simulink model "HoverLock"  (R2024b)
settings: Solver=ode15s  StartTime=0.0  StopTime=8  FixedStep=1/120  MaxStep=0.01  RelTol=1e-1
PreLoadFcn:
  | [aircraft, state] = astDehavillandBeaver();
  | thrustX = getCoefficient(aircraft,"CX","Propeller",Component="Propeller");
model workspace (MATLAB code in the model file + MAT data in the model file):
  inputs0.time = 0
  inputs0.signals(1).dimensions = 1
  inputs0.signals(1).values = -0.104711430294
  inputs0.signals(2).dimensions = 1
  inputs0.signals(2).values = -0.0698725229544
  inputs0.signals(3).dimensions = 1
  inputs0.signals(3).values = -0.000215042330254
  states.time = 0
  states.signals(1).values = 0
  states.signals(1).dimensions = 1
  states.signals(1).label = 'CSTATE'
  states.signals(1).blockName = 'asb6DOFAirframeTemplate/6DOF EOM/6DOF (Euler Angles)/xe,ye,ze'
  states.signals(1).stateName = 'Xe'
  states.signals(1).inReferencedModel = 0
  states.signals(1).sampleTime = [0 0]
  states.signals(2).values = 0
  states.signals(2).dimensions = 1
  states.signals(2).label = 'CSTATE'
  states.signals(2).blockName = 'asb6DOFAirframeTemplate/6DOF EOM/6DOF (Euler Angles)/xe,ye,ze'
  states.signals(2).stateName = 'Ye'
  states.signals(2).inReferencedModel = 0
  states.signals(2).sampleTime = [0 0]
  states.signals(3).values = -2202
  states.signals(3).dimensions = 1
  states.signals(3).label = 'CSTATE'
  states.signals(3).blockName = 'asb6DOFAirframeTemplate/6DOF EOM/6DOF (Euler Angles)/xe,ye,ze'
  states.signals(3).stateName = 'Ze'
  states.signals(3).inReferencedModel = 0
  states.signals(3).sampleTime = [0 0]
  states.signals(4).values = 0.128665353089
  states.signals(4).dimensions = 1
  states.signals(4).label = 'CSTATE'
  states.signals(4).blockName = 'asb6DOFAirframeTemplate/6DOF EOM/6DOF (Euler Angles)/Calculate DCM &
    | Euler Angles/phi
    | theta
    | psi'
  states.signals(4).stateName = 'phi'
  states.signals(4).inReferencedModel = 0
  states.signals(4).sampleTime = [0 0]
  states.signals(5).values = 0.259337659946
  states.signals(5).dimensions = 1
  states.signals(5).label = 'CSTATE'
  states.signals(5).blockName = 'asb6DOFAirframeTemplate/6DOF EOM/6DOF (Euler Angles)/Calculate DCM &
    | Euler Angles/phi
    | theta
    | psi'
  states.signals(5).stateName = 'theta'
  states.signals(5).inReferencedModel = 0
  states.signals(5).sampleTime = [0 0]
  states.signals(6).values = -0.178947917154
  states.signals(6).dimensions = 1
  states.signals(6).label = 'CSTATE'
  states.signals(6).blockName = 'asb6DOFAirframeTemplate/6DOF EOM/6DOF (Euler Angles)/Calculate DCM &
    | Euler Angles/phi
    | theta
    | psi'
  states.signals(6).stateName = 'psi'
  states.signals(6).inReferencedModel = 0
  states.signals(6).sampleTime = [0 0]
  states.signals(7).values = 36.9119692666
  states.signals(7).dimensions = 1
  states.signals(7).label = 'CSTATE'
  states.signals(7).blockName = 'asb6DOFAirframeTemplate/6DOF EOM/6DOF (Euler Angles)/ub,vb,wb'
  states.signals(7).stateName = 'Ubody'
  states.signals(7).inReferencedModel = 0
  states.signals(7).sampleTime = [0 0]
  states.signals(8).values = 8.10720863264
  states.signals(8).dimensions = 1
  states.signals(8).label = 'CSTATE'
  states.signals(8).blockName = 'asb6DOFAirframeTemplate/6DOF EOM/6DOF (Euler Angles)/ub,vb,wb'
  states.signals(8).stateName = 'Vbody'
  states.signals(8).inReferencedModel = 0
  states.signals(8).sampleTime = [0 0]
  states.signals(9).values = 8.82591882596
  states.signals(9).dimensions = 1
  states.signals(9).label = 'CSTATE'
  states.signals(9).blockName = 'asb6DOFAirframeTemplate/6DOF EOM/6DOF (Euler Angles)/ub,vb,wb'
  states.signals(9).stateName = 'Wbody'
  states.signals(9).inReferencedModel = 0
  states.signals(9).sampleTime = [0 0]
  states.signals(10).values = 0
  states.signals(10).dimensions = 1
  states.signals(10).label = 'CSTATE'
  states.signals(10).blockName = 'asb6DOFAirframeTemplate/6DOF EOM/6DOF (Euler Angles)/p,q,r '
  states.signals(10).stateName = 'p'
  states.signals(10).inReferencedModel = 0
  states.signals(10).sampleTime = [0 0]
  states.signals(11).values = 0
  states.signals(11).dimensions = 1
  states.signals(11).label = 'CSTATE'
  states.signals(11).blockName = 'asb6DOFAirframeTemplate/6DOF EOM/6DOF (Euler Angles)/p,q,r '
  states.signals(11).stateName = 'q'
  states.signals(11).inReferencedModel = 0
  states.signals(11).sampleTime = [0 0]
  states.signals(12).values = 0
  states.signals(12).dimensions = 1
  states.signals(12).label = 'CSTATE'
  states.signals(12).blockName = 'asb6DOFAirframeTemplate/6DOF EOM/6DOF (Euler Angles)/p,q,r '
  states.signals(12).stateName = 'r'
  states.signals(12).inReferencedModel = 0
  states.signals(12).sampleTime = [0 0]
  states.signals(13).values = [0 0]
  states.signals(13).dimensions = 2
  states.signals(13).label = 'CSTATE'
  states.signals(13).blockName = 'asb6DOFAirframeTemplate/Environment Model/Dryden Wind Turbulence Model 
    | (Continuous (+q +r))/Filters on velocities/Hwgw(s)/wg_p1'
  states.signals(13).stateName = ''
  states.signals(13).inReferencedModel = 0
  states.signals(13).sampleTime = [0 0]
  states.signals(14).values = [0 0]
  states.signals(14).dimensions = 2
  states.signals(14).label = 'CSTATE'
  states.signals(14).blockName = 'asb6DOFAirframeTemplate/Environment Model/Dryden Wind Turbulence Model 
    | (Continuous (+q +r))/Filters on velocities/Hwgw(s)/wg_p2'
  states.signals(14).stateName = ''
  states.signals(14).inReferencedModel = 0
  states.signals(14).sampleTime = [0 0]
  states.signals(15).values = [0 0]
  states.signals(15).dimensions = 2
  states.signals(15).label = 'CSTATE'
  states.signals(15).blockName = 'asb6DOFAirframeTemplate/Environment Model/Dryden Wind Turbulence Model 
    | (Continuous (+q +r))/Filters on velocities/Hvgw(s)/vg_p1'
  states.signals(15).stateName = ''
  states.signals(15).inReferencedModel = 0
  states.signals(15).sampleTime = [0 0]
  states.signals(16).values = [0 0]
  states.signals(16).dimensions = 2
  states.signals(16).label = 'CSTATE'
  states.signals(16).blockName = 'asb6DOFAirframeTemplate/Environment Model/Dryden Wind Turbulence Model 
    | (Continuous (+q +r))/Filters on velocities/Hvgw(s)/vgw_p2'
  states.signals(16).stateName = ''
  states.signals(16).inReferencedModel = 0
  states.signals(16).sampleTime = [0 0]
  states.signals(17).values = [0 0]
  states.signals(17).dimensions = 2
  states.signals(17).label = 'CSTATE'
  states.signals(17).blockName = 'asb6DOFAirframeTemplate/Environment Model/Dryden Wind Turbulence Model 
    | (Continuous (+q +r))/Filters on velocities/Hugw(s)/ug_p'
  states.signals(17).stateName = ''
  states.signals(17).inReferencedModel = 0
  states.signals(17).sampleTime = [0 0]
  states.signals(18).values = [0 0]
  states.signals(18).dimensions = 2
  states.signals(18).label = 'CSTATE'
  states.signals(18).blockName = 'asb6DOFAirframeTemplate/Environment Model/Dryden Wind Turbulence Model 
    | (Continuous (+q +r))/Filters on angular rates/Hrgw/rgw_p'
  states.signals(18).stateName = ''
  states.signals(18).inReferencedModel = 0
  states.signals(18).sampleTime = [0 0]
  states.signals(19).values = [0 0]
  states.signals(19).dimensions = 2
  states.signals(19).label = 'CSTATE'
  states.signals(19).blockName = 'asb6DOFAirframeTemplate/Environment Model/Dryden Wind Turbulence Model 
    | (Continuous (+q +r))/Filters on angular rates/Hqgw/qgw_p'
  states.signals(19).stateName = ''
  states.signals(19).inReferencedModel = 0
  states.signals(19).sampleTime = [0 0]
  states.signals(20).values = [0 0]
  states.signals(20).dimensions = 2
  states.signals(20).label = 'CSTATE'
  states.signals(20).blockName = 'asb6DOFAirframeTemplate/Environment Model/Dryden Wind Turbulence Model 
    | (Continuous (+q +r))/Filters on angular rates/Hpgw/pgw_p'
  states.signals(20).stateName = ''
  states.signals(20).inReferencedModel = 0
  states.signals(20).sampleTime = [0 0]
  states0.time = 0
  states0.signals(1).values = [0 0 -2202]
  states0.signals(1).dimensions = 3
  states0.signals(1).label = 'CSTATE'
  states0.signals(1).blockName = 'asb6DOFAirframeTemplate/6DOF EOM/6DOF (Euler Angles)/xe,ye,ze'
  states0.signals(1).stateName = ''
  states0.signals(1).inReferencedModel = 0
  states0.signals(1).sampleTime = [0 0]
  states0.signals(2).values = [0.128665353089 0.259337659946 -0.178947917154]
  states0.signals(2).dimensions = 3
  states0.signals(2).label = 'CSTATE'
  states0.signals(2).blockName = 'asb6DOFAirframeTemplate/6DOF EOM/6DOF (Euler Angles)/Calculate DCM &
    | Euler Angles/phi
    | theta
    | psi'
  states0.signals(2).stateName = ''
  states0.signals(2).inReferencedModel = 0
  states0.signals(2).sampleTime = [0 0]
  states0.signals(3).values = [36.9119692666 8.10720863264 8.82591882596]
  states0.signals(3).dimensions = 3
  states0.signals(3).label = 'CSTATE'
  states0.signals(3).blockName = 'asb6DOFAirframeTemplate/6DOF EOM/6DOF (Euler Angles)/ub,vb,wb'
  states0.signals(3).stateName = ''
  states0.signals(3).inReferencedModel = 0
  states0.signals(3).sampleTime = [0 0]
  states0.signals(4).values = [0 0 0]
  states0.signals(4).dimensions = 3
  states0.signals(4).label = 'CSTATE'
  states0.signals(4).blockName = 'asb6DOFAirframeTemplate/6DOF EOM/6DOF (Euler Angles)/p,q,r '
  states0.signals(4).stateName = ''
  states0.signals(4).inReferencedModel = 0
  states0.signals(4).sampleTime = [0 0]
  states0.signals(5).values = [0 0]
  states0.signals(5).dimensions = 2
  states0.signals(5).label = 'CSTATE'
  states0.signals(5).blockName = 'asb6DOFAirframeTemplate/Environment Model/Dryden Wind Turbulence Model 
    | (Continuous (+q +r))/Filters on velocities/Hwgw(s)/wg_p1'
  states0.signals(5).stateName = ''
  states0.signals(5).inReferencedModel = 0
  states0.signals(5).sampleTime = [0 0]
  states0.signals(6).values = [0 0]
  states0.signals(6).dimensions = 2
  states0.signals(6).label = 'CSTATE'
  states0.signals(6).blockName = 'asb6DOFAirframeTemplate/Environment Model/Dryden Wind Turbulence Model 
    | (Continuous (+q +r))/Filters on velocities/Hwgw(s)/wg_p2'
  states0.signals(6).stateName = ''
  states0.signals(6).inReferencedModel = 0
  states0.signals(6).sampleTime = [0 0]
  states0.signals(7).values = [0 0]
  states0.signals(7).dimensions = 2
  states0.signals(7).label = 'CSTATE'
  states0.signals(7).blockName = 'asb6DOFAirframeTemplate/Environment Model/Dryden Wind Turbulence Model 
    | (Continuous (+q +r))/Filters on velocities/Hvgw(s)/vg_p1'
  states0.signals(7).stateName = ''
  states0.signals(7).inReferencedModel = 0
  states0.signals(7).sampleTime = [0 0]
  states0.signals(8).values = [0 0]
  states0.signals(8).dimensions = 2
  states0.signals(8).label = 'CSTATE'
  states0.signals(8).blockName = 'asb6DOFAirframeTemplate/Environment Model/Dryden Wind Turbulence Model 
    | (Continuous (+q +r))/Filters on velocities/Hvgw(s)/vgw_p2'
  states0.signals(8).stateName = ''
  states0.signals(8).inReferencedModel = 0
  states0.signals(8).sampleTime = [0 0]
  states0.signals(9).values = [0 0]
  states0.signals(9).dimensions = 2
  states0.signals(9).label = 'CSTATE'
  states0.signals(9).blockName = 'asb6DOFAirframeTemplate/Environment Model/Dryden Wind Turbulence Model 
    | (Continuous (+q +r))/Filters on velocities/Hugw(s)/ug_p'
  states0.signals(9).stateName = ''
  states0.signals(9).inReferencedModel = 0
  states0.signals(9).sampleTime = [0 0]
  states0.signals(10).values = [0 0]
  states0.signals(10).dimensions = 2
  states0.signals(10).label = 'CSTATE'
  states0.signals(10).blockName = 'asb6DOFAirframeTemplate/Environment Model/Dryden Wind Turbulence Model 
    | (Continuous (+q +r))/Filters on angular rates/Hrgw/rgw_p'
  states0.signals(10).stateName = ''
  states0.signals(10).inReferencedModel = 0
  states0.signals(10).sampleTime = [0 0]
  states0.signals(11).values = [0 0]
  states0.signals(11).dimensions = 2
  states0.signals(11).label = 'CSTATE'
  states0.signals(11).blockName = 'asb6DOFAirframeTemplate/Environment Model/Dryden Wind Turbulence Model 
    | (Continuous (+q +r))/Filters on angular rates/Hqgw/qgw_p'
  states0.signals(11).stateName = ''
  states0.signals(11).inReferencedModel = 0
  states0.signals(11).sampleTime = [0 0]
  states0.signals(12).values = [0 0]
  states0.signals(12).dimensions = 2
  states0.signals(12).label = 'CSTATE'
  states0.signals(12).blockName = 'asb6DOFAirframeTemplate/Environment Model/Dryden Wind Turbulence Model 
    | (Continuous (+q +r))/Filters on angular rates/Hpgw/pgw_p'
  states0.signals(12).stateName = ''
  states0.signals(12).inReferencedModel = 0
  states0.signals(12).sampleTime = [0 0]
  other statements: initialize6DOFSkyHogg;
libraries: fl_lib x15, slpidlib x10, nesl_utility x3, simulink x3
settings Model: Creator=asus  LastModifiedBy=asus
settings SolverCC: AlgebraicLoopSolver=TrustRegion  AutoInsertRateTranBlk=on  InsertRTBMode=Never (minimum delay)  MinimalZcImpactIntegration=on  MaxZcPerStep=1
settings DataIOCC: ExternalInput=inputs0  InitialState=states  SaveFormat=Array  SaveOutput=off
settings OptimizationCC: EnhancedBackFolding=on  StrengthReduction=on  InitFltsAndDblsToZero=on  DifferentSizesBufferReuse=on
settings DebuggingCC: WriteAfterWriteMsg=DisableAll  AlgebraicLoopMsg=none  FcnCallInpInsideContextMsg=warning  UniqueDataStoreMsg=error  RootOutportRequireBusObject=none  StateNameClashWarn=warning  StrictBusMsg=ErrorOnBusTreatedAsVector  SFUnexpectedBacktrackingDiag=warning  SFNoUnconditionalDefaultTransitionDiag=warning  SFExecutionAtInitializationDiag=none  ArithmeticOperatorsInVariantConditions=warning
settings ModelReferenceCC: EnableRefExpFcnMdlSchedulingChecks=on  PropagateSignalLabelsOutOfModel=off
settings SFSimCC: SimUseLocalCustomCode=off
settings RTWCC: RTWUseLocalCustomCode=off  GPUComputeCapability=3.5  DLArmComputeVersion=19.05
settings CodeAppCC: StateflowObjectComments=on

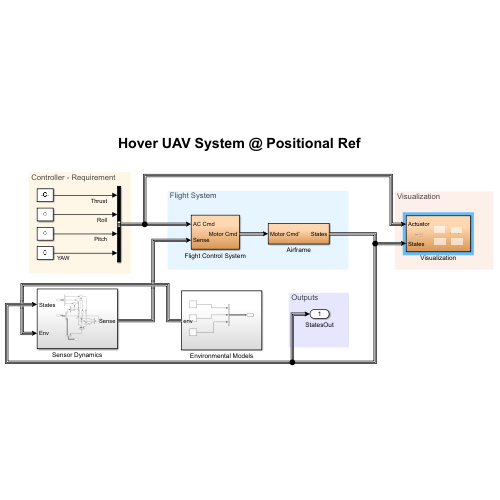
[thumbnail: Simulink's stored preview of the top-level diagram]
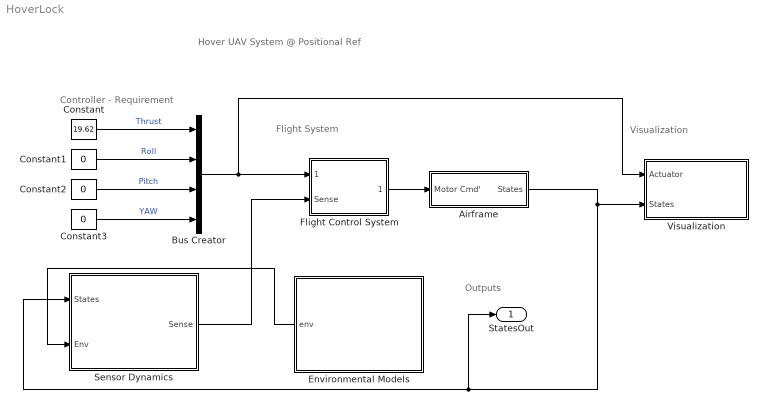
== system HoverLock ==
  note: Hover UAV System @ Positional Ref
  note: Flight System
  note: Controller - Requirement
  note: Visualization
  note: Outputs
  Airframe : Subsystem  VariantControl=eom3DOF
  Bus Creator : BusCreator  Inputs=4
  Constant : Constant  Value=19.62
  Constant1 : Constant  Value=0
  Constant2 : Constant  Value=0
  Constant3 : Constant  Value=0
  Environmental Models : Subsystem
  Flight Control System : Subsystem  VariantControl=aeroCONST
  Sensor Dynamics : Subsystem
  Visualization : Subsystem
  StatesOut : Outport  OutDataTypeStr=double  VectorParamsAs1DForOutWhenUnconnected=off
  wires:
  Constant/1 -> Bus Creator/1  "Thrust"
  Constant1/1 -> Bus Creator/2  "Roll"
  Constant2/1 -> Bus Creator/3  "Pitch"
  Airframe/1(States) -> Visualization/2(States), StatesOut/1, Sensor Dynamics/1(States)
  Environmental Models/1(env) -> Sensor Dynamics/2(Env)
  Constant3/1 -> Bus Creator/4  "YAW"
  Bus Creator/1 -> Visualization/1(Actuator), Flight Control System/1(AC Cmd)
  Flight Control System/1(Motor Cmd) -> Airframe/1(Motor Cmd')
  Sensor Dynamics/1(Sense) -> Flight Control System/2(Sense)

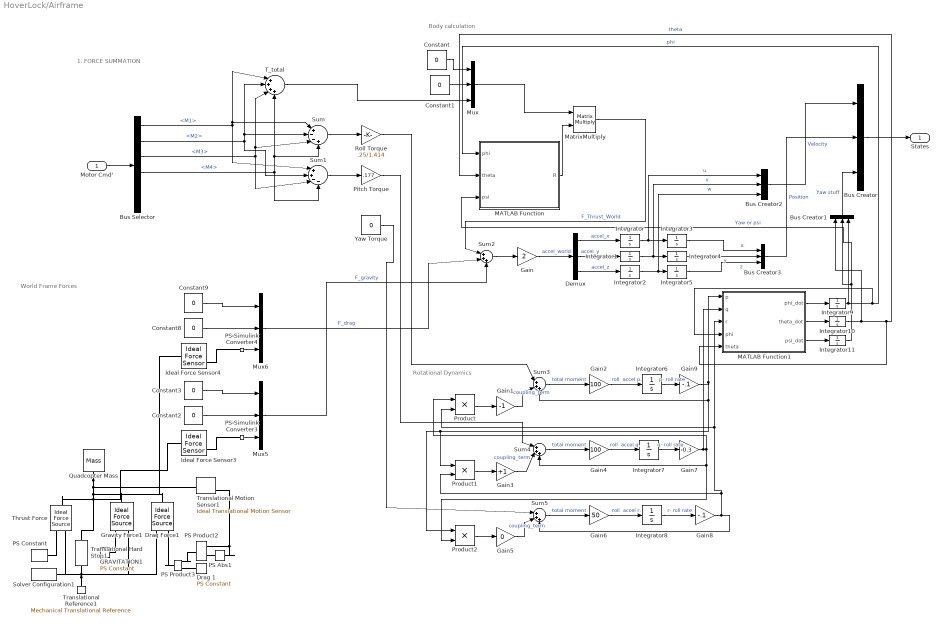
== system HoverLock/Airframe ==
  note: Body calculation
  note: Rotational Dynamics
  note: World Frame Forces
  note: 1. FORCE SUMMATION
  Motor Cmd' : Inport
  Bus Creator{,1..3} (4 alike) : BusCreator  Inputs=3
  Bus Selector : BusSelector  OutputSignals=M1,M2,M3,M4,theta,phi
  Constant : Constant  Value=0  VectorParams1D=off
  Constant1 : Constant  Value=0  VectorParams1D=off
  Constant{2..3,8..9} (4 alike) : Constant  Value=0
  Demux : Demux  Outputs=3
  Drag Force1 : fl_lib/Mechanical/Mechanical Sources/Ideal Force Source
  Drag 1 : fl_lib/Physical Signals/Sources/PS Constant  constant=-.5*1.225*1.1*0.006 N/(m/s)^2
  GRAVITATION1 : fl_lib/Physical Signals/Sources/PS Constant  constant=-9.81*.07 N
  Gain : Gain  Gain=2
  Gain1 : Gain  Gain=-1
  Gain2 : Gain  Gain=100
  Gain3 : Gain  Gain=+1
  Gain4 : Gain  Gain=100
  Gain5 : Gain  Gain=0
  Gain6 : Gain  Gain=50
  Gain7 : Gain  Gain=-0.3
  Gain8 : Gain  Gain=-.1
  Gain9 : Gain  Gain=-.1
  Gravity Force1 : fl_lib/Mechanical/Mechanical Sources/Ideal Force Source
  Ideal Force Sensor3 : fl_lib/Mechanical/Mechanical Sensors/Ideal Force Sensor
  Ideal Force Sensor4 : fl_lib/Mechanical/Mechanical Sensors/Ideal Force Sensor
  Integrator{,1..4,6..11} (11 alike) : Integrator
  Integrator5 : Integrator  InitialCondition=1
  MATLAB Function : MATLAB Function  TreatAsAtomicUnit=on
  MATLAB Function1 : MATLAB Function  TreatAsAtomicUnit=on
  MatrixMultiply : Product  Multiplication=Matrix(*)
  Mux : Mux  Inputs=3
  Mux5 : Mux  Inputs=3
  Mux6 : Mux  Inputs=3
  PS Abs1 : fl_lib/Physical Signals/Nonlinear Operators/PS Abs
      settings: InternalSimscapePortConfiguration="{\"Bottom\":[],\"Left\":[{\"id\":\"I\",\"label\":\"\",\"type\":\"input\"}],\"Right\":[{\"id\":\"O\",\"label\":\"\",\"type\":\"output\"}],\"Top\":[]}"
  PS Constant : fl_lib/Physical Signals/Sources/PS Constant  constant=19.62 N
  PS Product2 : fl_lib/Physical Signals/Functions/PS Product
  PS Product3 : fl_lib/Physical Signals/Functions/PS Product
  PS-Simulink Converter3 : nesl_utility/PS-Simulink Converter  PhysicalDomain=network_engine_domain  SubClassName=ps_output  LeftPortType=input  RightPortType=output  PseudoPeriodic=off  Frequencies=[]  VectorFormat=inherit  Unit=inherit  AffineConversion=off
  PS-Simulink Converter4 : nesl_utility/PS-Simulink Converter  PhysicalDomain=network_engine_domain  SubClassName=ps_output  LeftPortType=input  RightPortType=output  PseudoPeriodic=off  Frequencies=[]  VectorFormat=inherit  Unit=inherit  AffineConversion=off
  Pitch Torque : Gain  Gain=.177
  Product : Product
  Product1 : Product
  Product2 : Product
  Quadcopter Mass : fl_lib/Mechanical/Translational Elements/Mass  mass=.07 kg  num_ports=foundation.enum.numPorts2.one  v_specify=off  v_priority=High  v=0 m/s  v_nominal_specify=off  v_nominal_value=1  v_nominal_unit=m/s  f_specify=off  f_priority=None  f=0 N  f_nominal_specify=off  f_nominal_value=1  f_nominal_unit=N
  Roll Torque : Gain  Gain=.25/1.414
  Solver Configuration1 : nesl_utility/Solver Configuration  PhysicalDomain=network_engine_domain  SubClassName=solver  LeftPortType=input  RightPortType=generic  Tones=[]  Harmonics=[]  SimulateNoise=off  Profile=off  UseLocalSampling=off  EnableSwitchedLinearOptims=on  FrequencyDomain=off  UseCCode=off  RelTol=0.001  AbsTol=0.001  MinStep=1e-09  ToWorkspace=off  RevertToSquareIcSolve=off  NumHomotopyIterations=100  PhasorMode=off  PhasorModeNumHarmonics=1  ConsistencySolver=NEWTON_XTOL_AFTER_FTOL  IndexReductionMethod=DerivativeReplacement  DoDC=off  ResidualTolerance=1e-09  ConsistencyTolSource=GLOBAL  ConsistencyAbsTol=0.001  ConsistencyRelTol=0.001  ConsistencyTolFactor=0.001  UseLocalSolver=off  LocalSolverChoice=NE_BACKWARD_EULER_ADVANCER  ResolveIndetEquations=on  FunctionEvalNumThread=1  LocalSolverSampleTime=0.001  DoFixedCost=off  MaxNonlinIter=3  MaxModeIter=2  ComputeImpulses=off  ImpulseIterations=2  LinearAlgebra=auto  LinearAlgebraNumThread=0  EquationFormulation=NE_TIME_EF  DelaysMemoryBudget=1024  AutomaticFiltering=on  FilteringTimeConstant=0.001  PartitionStorageMethod=AS_NEEDED  PartitionMemoryBudget=1024  PartitionMethod=ROBUST  MultibodyUseLocalSolver=off  MultibodyLocalSolverChoice=ODE1  MultibodyLocalSolverSampleTime=0.001
  Sum : Sum  Inputs=|+--+
  Sum1 : Sum  Inputs=|++--
  Sum{2..5} (4 alike) : Sum  Inputs=|+++
  T_total : Sum  Inputs=|++++
  Thrust Force : fl_lib/Mechanical/Mechanical Sources/Ideal Force Source
  Translational Motion Sensor1 : fl_lib/Mechanical/Mechanical Sensors/Ideal Translational Motion Sensor  reference=foundation.enum.MeasurementReference.absolute  acceleration_port=false  velocity_port=true  position_port=true  offset=0 m
      settings: InternalSimscapePortConfiguration="{\"Bottom\":[],\"Left\":[{\"id\":\"R\",\"label\":\"R\",\"type\":\"foundation.mechanical.translational.translational\"}],\"Right\":[{\"id\":\"V\",\"label\":\"V\",\"type\":\"output\"},{\"id\":\"P\",\"label\":\"P\",\"type\":\"output\"}],\"Top\":[]}"
  Translational Reference1 : fl_lib/Mechanical/Translational Elements/Mechanical Translational Reference
  Translational Hard Stop1 : fl_lib/Mechanical/Translational Elements/Translational Hard Stop  upper_bnd=inf m  lower_bnd=0 m  model=simscape.enum.hardstop.smooth  stiff_up=1e6 N/m  stiff_low=270 N/m  D_up=150 N*s/m  D_low=150 N*s/m  transition=0.1 mm  coeff_rest=0.7  v_tol=0.001 m/s  f_tol=0.001 N  v_specify=off  v_priority=None  v=0 m/s  v_nominal_specify=off  v_nominal_value=1  v_nominal_unit=m/s  f_specify=off  f_priority=None  f=0 N  f_nominal_specify=off  f_nominal_value=1  f_nominal_unit=N  x_specify=off  x_priority=High  x=0 m  x_nominal_specify=off  x_nominal_value=1  x_nominal_unit=m  M_specify=off  M_priority=None  M=0
  Yaw Torque : Constant  Value=0
  States : Outport
  wires:
  Motor Cmd'/1 -> Bus Selector/1
  Bus Selector/2 -> Sum/2, T_total/2, Sum1/2  "<M2>"
  Bus Selector/3 -> Sum1/3, T_total/3, Sum/3  "<M3>"
  Bus Selector/4 -> Sum1/4, Sum/4, T_total/4  "<M4>"
  Bus Selector/1 -> Sum/1, T_total/1, Sum1/1  "<M1>"
  Sum/1 -> Roll Torque/1
  Sum1/1 -> Pitch Torque/1
  Constant/1 -> Mux/1
  Constant1/1 -> Mux/2
  T_total/1 -> Mux/3
  Mux/1 -> MatrixMultiply/1
  MATLAB Function/1(R) -> MatrixMultiply/2
  MatrixMultiply/1 -> Sum2/1  "F_Thrust_World"
  Sum2/1 -> Gain/1
  Gain/1 -> Demux/1  "accel_world"
  Demux/1 -> Integrator/1  "accel_x"
  Demux/2 -> Integrator1/1  "accel_y"
  Demux/3 -> Integrator2/1  "accel_z"
  Integrator/1 -> Bus Creator2/1, Integrator3/1  "u"
  Integrator1/1 -> Bus Creator2/2, Integrator4/1  "v"
  Integrator2/1 -> Bus Creator2/3, Integrator5/1  "w"
  Integrator3/1 -> Bus Creator3/1  "x"
  Integrator4/1 -> Bus Creator3/2  "y"
  Integrator5/1 -> Bus Creator3/3  "z"
  Product/1 -> Gain1/1
  Gain1/1 -> Sum3/2  "coupling_term"
  Sum3/1 -> Gain2/1  "total moment"
  Gain2/1 -> Integrator6/1  "roll  accel p."
  Integrator6/1 -> Gain9/1  "p- roll rate"
  Sum4/1 -> Gain4/1  "total moment"
  Gain3/1 -> Sum4/2  "coupling_term"
  Product1/1 -> Gain3/1
  Product2/1 -> Gain5/1
  Gain5/1 -> Sum5/2  "coupling_term"
  Sum5/1 -> Gain6/1  "total moment"
  Gain6/1 -> Integrator8/1  "roll  accel r."
  Integrator8/1 -> Gain8/1  "r- roll rate"
  Roll Torque/1 -> Sum3/1
  Pitch Torque/1 -> Sum4/1
  Yaw Torque/1 -> Sum5/1
  MATLAB Function1/1(phi_dot) -> Integrator9/1
  MATLAB Function1/2(theta_dot) -> Integrator10/1
  MATLAB Function1/3(psi_dot) -> Integrator11/1
  Integrator9/1 -> MATLAB Function1/4(phi), MATLAB Function/1(phi), Bus Creator1/3  "phi"
  Integrator10/1 -> Bus Creator1/1, MATLAB Function1/5(theta), MATLAB Function/2(theta)  "theta"
  Integrator11/1 -> Bus Creator1/2, MATLAB Function/3(psi)  "Yaw or psi"
  Bus Creator/1 -> States/1
  Bus Creator1/1 -> Bus Creator/3  "Yaw stuff"
  Gain7/1 -> Product2/2, Sum4/3, Product/1, MATLAB Function1/2(q)
  Integrator7/1 -> Gain7/1  "q- roll rate"
  Gain8/1 -> Sum5/3, Product1/2, Product/2, MATLAB Function1/3(r)
  Gain9/1 -> Product2/1, Product1/1, Sum3/3, MATLAB Function1/1(p)
  Gain4/1 -> Integrator7/1  "roll  accel q."
  Constant8/1 -> Mux6/2
  Mux6/1 -> Sum2/2  "F_drag"
  PS-Simulink Converter4/1 -> Mux6/3
  Constant9/1 -> Mux6/1
  Constant3/1 -> Mux5/1
  PS-Simulink Converter3/1 -> Mux5/3
  Constant2/1 -> Mux5/2
  Mux5/1 -> Sum2/3  "F_gravity"
  Bus Creator2/1 -> Bus Creator/1  "Velocity"
  Bus Creator3/1 -> Bus Creator/2  "Position"
  connections:
  Translational Reference1/LConn1 -- Drag Force1/RConn2 -- Gravity Force1/RConn2 -- Translational Hard Stop1/RConn1 -- Thrust Force/RConn2 -- Solver Configuration1/RConn1
  PS Abs1/LConn1 -- Translational Motion Sensor1/RConn1 -- PS Product2/LConn1
  Quadcopter Mass/LConn1 -- Translational Motion Sensor1/LConn1 -- Ideal Force Sensor4/LConn1 -- Drag Force1/LConn1 -- Ideal Force Sensor3/LConn1 -- Gravity Force1/LConn1 -- Thrust Force/LConn1 -- Translational Hard Stop1/LConn1
  PS Product3/RConn1 -- Drag Force1/RConn1
  PS Constant/RConn1 -- Thrust Force/RConn1
  PS Product3/LConn1 -- PS Product2/RConn1
  Gravity Force1/RConn1 -- GRAVITATION1/RConn1
  PS Abs1/RConn1 -- PS Product2/LConn2
  Drag 1/RConn1 -- PS Product3/LConn2
  Ideal Force Sensor4/RConn2 -- PS-Simulink Converter4/LConn1
  Ideal Force Sensor3/RConn2 -- PS-Simulink Converter3/LConn1

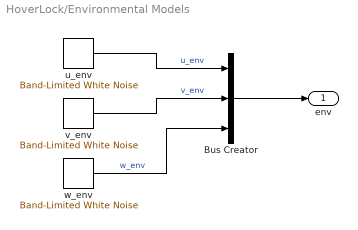
== system HoverLock/Environmental Models ==
  Bus Creator : BusCreator  Inputs=3
  u_env : simulink/Sources/Band-Limited White Noise  Cov=7  Ts=.08  seed=94864
  v_env : simulink/Sources/Band-Limited White Noise  Cov=7  Ts=.7  seed=12154
  w_env : simulink/Sources/Band-Limited White Noise  Cov=.7  Ts=.08  seed=45681
  env : Outport
  wires:
  u_env/1 -> Bus Creator/1  "u_env"
  v_env/1 -> Bus Creator/2  "v_env"
  w_env/1 -> Bus Creator/3  "w_env"
  Bus Creator/1 -> env/1

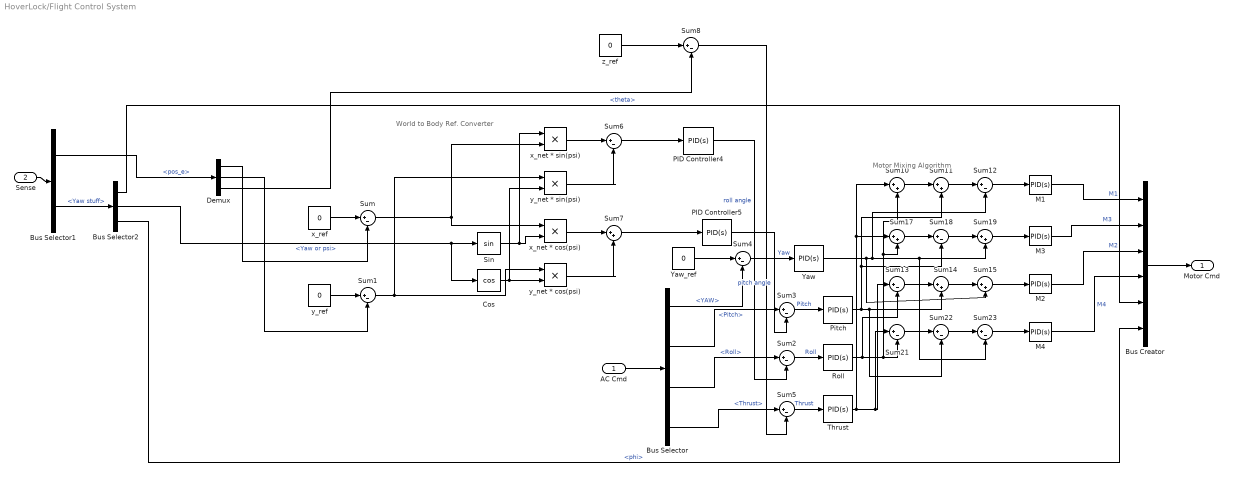
== system HoverLock/Flight Control System ==
  note: Motor Mixing Algorithm
  note: World to Body Ref. Converter
  AC Cmd : Inport
  Sense : Inport  Port=2
  Bus Creator : BusCreator  Inputs=6
  Bus Selector : BusSelector  OutputSignals=YAW,Pitch,Roll,Thrust
  Bus Selector1 : BusSelector  OutputSignals=pos_e,Yaw stuff
  Bus Selector2 : BusSelector  OutputSignals=theta,Yaw or psi,phi
  Cos : Trigonometry  Operator=cos
  Demux : Demux  Outputs=3
  M{1..4} (4 alike) : slpidlib/PID Controller  Controller=PID  Form=Parallel  TimeDomain=Continuous-time  UseExternalTs=off  SampleTime=-1  IntegratorMethod=Forward Euler  FilterMethod=Forward Euler  ControllerParametersSource=internal  P=1  I=1  UseKiTs=off  D=0  UseExternalDerivativeSource=off  N=100  UseFilter=on  TunerSelectOption=Transfer Function Based (PID Tuner App)  InitialConditionSource=internal  InitialConditionForIntegrator=0  InitialConditionForFilter=0  DifferentiatorICPrevScaledInput=0  ExternalReset=none  TrackingMode=off  Kt=1  LimitOutput=off  SatLimitsSource=internal  UpperSaturationLimit=inf  LowerSaturationLimit=-inf  LinearizeAsGain=on  AntiWindupMode=none  Kb=1  LimitIntegrator=off  UpperIntegratorSaturationLimit=inf  LowerIntegratorSaturationLimit=-inf  POutMin=[]  POutMax=[]  IOutMin=[]  IOutMax=[]  DOutMin=[]  DOutMax=[]  NOutMin=[]  NOutMax=[]  SumOutMin=[]  SumOutMax=[]  SaturationOutMin=[]  SaturationOutMax=[]  PParamMin=[]  PParamMax=[]  IParamMin=[]  IParamMax=[]  DParamMin=[]  DParamMax=[]  NParamMin=[]  NParamMax=[]  KbParamMin=[]  KbParamMax=[]  KtParamMin=[]  KtParamMax=[]  KbOutMin=[]  KbOutMax=[]  KtOutMin=[]  KtOutMax=[]  IntegratorOutMin=[]  IntegratorOutMax=[]  FilterOutMin=[]  FilterOutMax=[]  SumI1OutMin=[]  SumI1OutMax=[]  SumI2OutMin=[]  SumI2OutMax=[]  SumI3OutMin=[]  SumI3OutMax=[]  SumI4OutMin=[]  SumI4OutMax=[]  SumDOutMin=[]  SumDOutMax=[]  DifferentiatorOutMin=[]  DifferentiatorOutMax=[]  FilterDiffOutCoefMin=[]  FilterDiffOutCoefMax=[]  ReciprocalOutMin=[]  ReciprocalOutMax=[]  SumDenOutMin=[]  SumDenOutMax=[]  SumNumOutMin=[]  SumNumOutMax=[]  DivideOutMin=[]  DivideOutMax=[]  UdiffTsProdOutMin=[]  UdiffTsProdOutMax=[]  NTsProdOutMin=[]  NTsProdOutMax=[]  UintegralTsProdOutMin=[]  UintegralTsProdOutMax=[]  UngainTsProdOutMin=[]  UngainTsProdOutMax=[]  ClampingZeroOutDataTypeStr=Inherit: Inherit via back propagation  ClampingZeroOutMin=[]  ClampingZeroOutMax=[]  FilterDenConstantOutDataTypeStr=Inherit: Inherit via back propagation  FilterDenConstantOutMin=[]  FilterDenConstantOutMax=[]  PCopyOutDataTypeStr=Inherit: Inherit via back propagation  PCopyOutMin=[]  PCopyOutMax=[]  NCopyOutDataTypeStr=Inherit: Inherit via back propagation  NCopyOutMin=[]  NCopyOutMax=[]  IntegratorContinuousStateAttributes=''  IntegratorStateMustResolveToSignalObject=off  IntegratorRTWStateStorageClass=Auto  FilterContinuousStateAttributes=''  FilterStateMustResolveToSignalObject=off  FilterRTWStateStorageClass=Auto  ParallelPVariant=InternalParameters  IdealPVariant=Disabled  IVariant=InternalParameters  DVariant=InternalParameters  IntegratorVariant=Continuous  SatVariant=Disabled  AWVariant=Passthrough  PCopyVariant=Disabled  TRVariant=Disabled  FdbkBlocksVariant=Forward  IdealPFdbkVariant=Disabled  SatFdbkVariant=Disabled  DerivativeFilterVariant=ContFilter  NVariant=InternalParameters  NCopyVariant=Disabled  FilterICVariant=InternalICsFilter  IntegratorICVariant=InternalICs  ExternalResetVariant=Disabled  TRSumVariant=Passthrough  SumFdbkVariant=Disabled  SumVariant=Sum_PID  TsampFilterVariant=InternalTs  TsampNgainVariant=Passthrough  TsampIntegralVariant=Disabled_SignalSpec  ExternalSaturationOutDataTypeStr=Inherit: Same as second input  DerivativeSourceVariant=ErrorSignal  PreIntVariant=InternalPreInt
  PID Controller4 : slpidlib/PID Controller  Controller=PID  Form=Parallel  TimeDomain=Continuous-time  UseExternalTs=off  SampleTime=-1  IntegratorMethod=Forward Euler  FilterMethod=Forward Euler  ControllerParametersSource=internal  P=1  I=1  UseKiTs=off  D=0  UseExternalDerivativeSource=off  N=100  UseFilter=on  TunerSelectOption=Transfer Function Based (PID Tuner App)  InitialConditionSource=internal  InitialConditionForIntegrator=0  InitialConditionForFilter=0  DifferentiatorICPrevScaledInput=0  ExternalReset=none  TrackingMode=off  Kt=1  LimitOutput=off  SatLimitsSource=internal  UpperSaturationLimit=inf  LowerSaturationLimit=-inf  LinearizeAsGain=on  AntiWindupMode=none  Kb=1  LimitIntegrator=off  UpperIntegratorSaturationLimit=inf  LowerIntegratorSaturationLimit=-inf  POutMin=[]  POutMax=[]  IOutMin=[]  IOutMax=[]  DOutMin=[]  DOutMax=[]  NOutMin=[]  NOutMax=[]  SumOutMin=[]  SumOutMax=[]  SaturationOutMin=[]  SaturationOutMax=[]  PParamMin=[]  PParamMax=[]  IParamMin=[]  IParamMax=[]  DParamMin=[]  DParamMax=[]  NParamMin=[]  NParamMax=[]  KbParamMin=[]  KbParamMax=[]  KtParamMin=[]  KtParamMax=[]  KbOutMin=[]  KbOutMax=[]  KtOutMin=[]  KtOutMax=[]  IntegratorOutMin=[]  IntegratorOutMax=[]  FilterOutMin=[]  FilterOutMax=[]  SumI1OutMin=[]  SumI1OutMax=[]  SumI2OutMin=[]  SumI2OutMax=[]  SumI3OutMin=[]  SumI3OutMax=[]  SumI4OutMin=[]  SumI4OutMax=[]  SumDOutMin=[]  SumDOutMax=[]  DifferentiatorOutMin=[]  DifferentiatorOutMax=[]  FilterDiffOutCoefMin=[]  FilterDiffOutCoefMax=[]  ReciprocalOutMin=[]  ReciprocalOutMax=[]  SumDenOutMin=[]  SumDenOutMax=[]  SumNumOutMin=[]  SumNumOutMax=[]  DivideOutMin=[]  DivideOutMax=[]  UdiffTsProdOutMin=[]  UdiffTsProdOutMax=[]  NTsProdOutMin=[]  NTsProdOutMax=[]  UintegralTsProdOutMin=[]  UintegralTsProdOutMax=[]  UngainTsProdOutMin=[]  UngainTsProdOutMax=[]  ClampingZeroOutDataTypeStr=Inherit: Inherit via back propagation  ClampingZeroOutMin=[]  ClampingZeroOutMax=[]  FilterDenConstantOutDataTypeStr=Inherit: Inherit via back propagation  FilterDenConstantOutMin=[]  FilterDenConstantOutMax=[]  PCopyOutDataTypeStr=Inherit: Inherit via back propagation  PCopyOutMin=[]  PCopyOutMax=[]  NCopyOutDataTypeStr=Inherit: Inherit via back propagation  NCopyOutMin=[]  NCopyOutMax=[]  IntegratorContinuousStateAttributes=''  IntegratorStateMustResolveToSignalObject=off  IntegratorRTWStateStorageClass=Auto  FilterContinuousStateAttributes=''  FilterStateMustResolveToSignalObject=off  FilterRTWStateStorageClass=Auto  ParallelPVariant=InternalParameters  IdealPVariant=Disabled  IVariant=InternalParameters  DVariant=InternalParameters  IntegratorVariant=Continuous  SatVariant=Disabled  AWVariant=Passthrough  PCopyVariant=Disabled  TRVariant=Disabled  FdbkBlocksVariant=Forward  IdealPFdbkVariant=Disabled  SatFdbkVariant=Disabled  DerivativeFilterVariant=ContFilter  NVariant=InternalParameters  NCopyVariant=Disabled  FilterICVariant=InternalICsFilter  IntegratorICVariant=InternalICs  ExternalResetVariant=Disabled  TRSumVariant=Passthrough  SumFdbkVariant=Disabled  SumVariant=Sum_PID  TsampFilterVariant=InternalTs  TsampNgainVariant=Passthrough  TsampIntegralVariant=Disabled_SignalSpec  ExternalSaturationOutDataTypeStr=Inherit: Same as second input  DerivativeSourceVariant=ErrorSignal  PreIntVariant=InternalPreInt
  PID Controller5 : slpidlib/PID Controller  Controller=PID  Form=Parallel  TimeDomain=Continuous-time  UseExternalTs=off  SampleTime=-1  IntegratorMethod=Forward Euler  FilterMethod=Forward Euler  ControllerParametersSource=internal  P=1  I=1  UseKiTs=off  D=0  UseExternalDerivativeSource=off  N=100  UseFilter=on  TunerSelectOption=Transfer Function Based (PID Tuner App)  InitialConditionSource=internal  InitialConditionForIntegrator=0  InitialConditionForFilter=0  DifferentiatorICPrevScaledInput=0  ExternalReset=none  TrackingMode=off  Kt=1  LimitOutput=off  SatLimitsSource=internal  UpperSaturationLimit=inf  LowerSaturationLimit=-inf  LinearizeAsGain=on  AntiWindupMode=none  Kb=1  LimitIntegrator=off  UpperIntegratorSaturationLimit=inf  LowerIntegratorSaturationLimit=-inf  POutMin=[]  POutMax=[]  IOutMin=[]  IOutMax=[]  DOutMin=[]  DOutMax=[]  NOutMin=[]  NOutMax=[]  SumOutMin=[]  SumOutMax=[]  SaturationOutMin=[]  SaturationOutMax=[]  PParamMin=[]  PParamMax=[]  IParamMin=[]  IParamMax=[]  DParamMin=[]  DParamMax=[]  NParamMin=[]  NParamMax=[]  KbParamMin=[]  KbParamMax=[]  KtParamMin=[]  KtParamMax=[]  KbOutMin=[]  KbOutMax=[]  KtOutMin=[]  KtOutMax=[]  IntegratorOutMin=[]  IntegratorOutMax=[]  FilterOutMin=[]  FilterOutMax=[]  SumI1OutMin=[]  SumI1OutMax=[]  SumI2OutMin=[]  SumI2OutMax=[]  SumI3OutMin=[]  SumI3OutMax=[]  SumI4OutMin=[]  SumI4OutMax=[]  SumDOutMin=[]  SumDOutMax=[]  DifferentiatorOutMin=[]  DifferentiatorOutMax=[]  FilterDiffOutCoefMin=[]  FilterDiffOutCoefMax=[]  ReciprocalOutMin=[]  ReciprocalOutMax=[]  SumDenOutMin=[]  SumDenOutMax=[]  SumNumOutMin=[]  SumNumOutMax=[]  DivideOutMin=[]  DivideOutMax=[]  UdiffTsProdOutMin=[]  UdiffTsProdOutMax=[]  NTsProdOutMin=[]  NTsProdOutMax=[]  UintegralTsProdOutMin=[]  UintegralTsProdOutMax=[]  UngainTsProdOutMin=[]  UngainTsProdOutMax=[]  ClampingZeroOutDataTypeStr=Inherit: Inherit via back propagation  ClampingZeroOutMin=[]  ClampingZeroOutMax=[]  FilterDenConstantOutDataTypeStr=Inherit: Inherit via back propagation  FilterDenConstantOutMin=[]  FilterDenConstantOutMax=[]  PCopyOutDataTypeStr=Inherit: Inherit via back propagation  PCopyOutMin=[]  PCopyOutMax=[]  NCopyOutDataTypeStr=Inherit: Inherit via back propagation  NCopyOutMin=[]  NCopyOutMax=[]  IntegratorContinuousStateAttributes=''  IntegratorStateMustResolveToSignalObject=off  IntegratorRTWStateStorageClass=Auto  FilterContinuousStateAttributes=''  FilterStateMustResolveToSignalObject=off  FilterRTWStateStorageClass=Auto  ParallelPVariant=InternalParameters  IdealPVariant=Disabled  IVariant=InternalParameters  DVariant=InternalParameters  IntegratorVariant=Continuous  SatVariant=Disabled  AWVariant=Passthrough  PCopyVariant=Disabled  TRVariant=Disabled  FdbkBlocksVariant=Forward  IdealPFdbkVariant=Disabled  SatFdbkVariant=Disabled  DerivativeFilterVariant=ContFilter  NVariant=InternalParameters  NCopyVariant=Disabled  FilterICVariant=InternalICsFilter  IntegratorICVariant=InternalICs  ExternalResetVariant=Disabled  TRSumVariant=Passthrough  SumFdbkVariant=Disabled  SumVariant=Sum_PID  TsampFilterVariant=InternalTs  TsampNgainVariant=Passthrough  TsampIntegralVariant=Disabled_SignalSpec  ExternalSaturationOutDataTypeStr=Inherit: Same as second input  DerivativeSourceVariant=ErrorSignal  PreIntVariant=InternalPreInt
  "Pitch " : slpidlib/PID Controller  Controller=PID  Form=Parallel  TimeDomain=Continuous-time  UseExternalTs=off  SampleTime=-1  IntegratorMethod=Forward Euler  FilterMethod=Forward Euler  ControllerParametersSource=internal  P=1  I=1  UseKiTs=off  D=0  UseExternalDerivativeSource=off  N=100  UseFilter=on  TunerSelectOption=Transfer Function Based (PID Tuner App)  InitialConditionSource=internal  InitialConditionForIntegrator=0  InitialConditionForFilter=0  DifferentiatorICPrevScaledInput=0  ExternalReset=none  TrackingMode=off  Kt=1  LimitOutput=off  SatLimitsSource=internal  UpperSaturationLimit=inf  LowerSaturationLimit=-inf  LinearizeAsGain=on  AntiWindupMode=none  Kb=1  LimitIntegrator=off  UpperIntegratorSaturationLimit=inf  LowerIntegratorSaturationLimit=-inf  POutMin=[]  POutMax=[]  IOutMin=[]  IOutMax=[]  DOutMin=[]  DOutMax=[]  NOutMin=[]  NOutMax=[]  SumOutMin=[]  SumOutMax=[]  SaturationOutMin=[]  SaturationOutMax=[]  PParamMin=[]  PParamMax=[]  IParamMin=[]  IParamMax=[]  DParamMin=[]  DParamMax=[]  NParamMin=[]  NParamMax=[]  KbParamMin=[]  KbParamMax=[]  KtParamMin=[]  KtParamMax=[]  KbOutMin=[]  KbOutMax=[]  KtOutMin=[]  KtOutMax=[]  IntegratorOutMin=[]  IntegratorOutMax=[]  FilterOutMin=[]  FilterOutMax=[]  SumI1OutMin=[]  SumI1OutMax=[]  SumI2OutMin=[]  SumI2OutMax=[]  SumI3OutMin=[]  SumI3OutMax=[]  SumI4OutMin=[]  SumI4OutMax=[]  SumDOutMin=[]  SumDOutMax=[]  DifferentiatorOutMin=[]  DifferentiatorOutMax=[]  FilterDiffOutCoefMin=[]  FilterDiffOutCoefMax=[]  ReciprocalOutMin=[]  ReciprocalOutMax=[]  SumDenOutMin=[]  SumDenOutMax=[]  SumNumOutMin=[]  SumNumOutMax=[]  DivideOutMin=[]  DivideOutMax=[]  UdiffTsProdOutMin=[]  UdiffTsProdOutMax=[]  NTsProdOutMin=[]  NTsProdOutMax=[]  UintegralTsProdOutMin=[]  UintegralTsProdOutMax=[]  UngainTsProdOutMin=[]  UngainTsProdOutMax=[]  ClampingZeroOutDataTypeStr=Inherit: Inherit via back propagation  ClampingZeroOutMin=[]  ClampingZeroOutMax=[]  FilterDenConstantOutDataTypeStr=Inherit: Inherit via back propagation  FilterDenConstantOutMin=[]  FilterDenConstantOutMax=[]  PCopyOutDataTypeStr=Inherit: Inherit via back propagation  PCopyOutMin=[]  PCopyOutMax=[]  NCopyOutDataTypeStr=Inherit: Inherit via back propagation  NCopyOutMin=[]  NCopyOutMax=[]  IntegratorContinuousStateAttributes=''  IntegratorStateMustResolveToSignalObject=off  IntegratorRTWStateStorageClass=Auto  FilterContinuousStateAttributes=''  FilterStateMustResolveToSignalObject=off  FilterRTWStateStorageClass=Auto  ParallelPVariant=InternalParameters  IdealPVariant=Disabled  IVariant=InternalParameters  DVariant=InternalParameters  IntegratorVariant=Continuous  SatVariant=Disabled  AWVariant=Passthrough  PCopyVariant=Disabled  TRVariant=Disabled  FdbkBlocksVariant=Forward  IdealPFdbkVariant=Disabled  SatFdbkVariant=Disabled  DerivativeFilterVariant=ContFilter  NVariant=InternalParameters  NCopyVariant=Disabled  FilterICVariant=InternalICsFilter  IntegratorICVariant=InternalICs  ExternalResetVariant=Disabled  TRSumVariant=Passthrough  SumFdbkVariant=Disabled  SumVariant=Sum_PID  TsampFilterVariant=InternalTs  TsampNgainVariant=Passthrough  TsampIntegralVariant=Disabled_SignalSpec  ExternalSaturationOutDataTypeStr=Inherit: Same as second input  DerivativeSourceVariant=ErrorSignal  PreIntVariant=InternalPreInt
  Roll : slpidlib/PID Controller  Controller=PID  Form=Parallel  TimeDomain=Continuous-time  UseExternalTs=off  SampleTime=-1  IntegratorMethod=Forward Euler  FilterMethod=Forward Euler  ControllerParametersSource=internal  P=1  I=1  UseKiTs=off  D=0  UseExternalDerivativeSource=off  N=100  UseFilter=on  TunerSelectOption=Transfer Function Based (PID Tuner App)  InitialConditionSource=internal  InitialConditionForIntegrator=0  InitialConditionForFilter=0  DifferentiatorICPrevScaledInput=0  ExternalReset=none  TrackingMode=off  Kt=1  LimitOutput=off  SatLimitsSource=internal  UpperSaturationLimit=inf  LowerSaturationLimit=-inf  LinearizeAsGain=on  AntiWindupMode=none  Kb=1  LimitIntegrator=off  UpperIntegratorSaturationLimit=inf  LowerIntegratorSaturationLimit=-inf  POutMin=[]  POutMax=[]  IOutMin=[]  IOutMax=[]  DOutMin=[]  DOutMax=[]  NOutMin=[]  NOutMax=[]  SumOutMin=[]  SumOutMax=[]  SaturationOutMin=[]  SaturationOutMax=[]  PParamMin=[]  PParamMax=[]  IParamMin=[]  IParamMax=[]  DParamMin=[]  DParamMax=[]  NParamMin=[]  NParamMax=[]  KbParamMin=[]  KbParamMax=[]  KtParamMin=[]  KtParamMax=[]  KbOutMin=[]  KbOutMax=[]  KtOutMin=[]  KtOutMax=[]  IntegratorOutMin=[]  IntegratorOutMax=[]  FilterOutMin=[]  FilterOutMax=[]  SumI1OutMin=[]  SumI1OutMax=[]  SumI2OutMin=[]  SumI2OutMax=[]  SumI3OutMin=[]  SumI3OutMax=[]  SumI4OutMin=[]  SumI4OutMax=[]  SumDOutMin=[]  SumDOutMax=[]  DifferentiatorOutMin=[]  DifferentiatorOutMax=[]  FilterDiffOutCoefMin=[]  FilterDiffOutCoefMax=[]  ReciprocalOutMin=[]  ReciprocalOutMax=[]  SumDenOutMin=[]  SumDenOutMax=[]  SumNumOutMin=[]  SumNumOutMax=[]  DivideOutMin=[]  DivideOutMax=[]  UdiffTsProdOutMin=[]  UdiffTsProdOutMax=[]  NTsProdOutMin=[]  NTsProdOutMax=[]  UintegralTsProdOutMin=[]  UintegralTsProdOutMax=[]  UngainTsProdOutMin=[]  UngainTsProdOutMax=[]  ClampingZeroOutDataTypeStr=Inherit: Inherit via back propagation  ClampingZeroOutMin=[]  ClampingZeroOutMax=[]  FilterDenConstantOutDataTypeStr=Inherit: Inherit via back propagation  FilterDenConstantOutMin=[]  FilterDenConstantOutMax=[]  PCopyOutDataTypeStr=Inherit: Inherit via back propagation  PCopyOutMin=[]  PCopyOutMax=[]  NCopyOutDataTypeStr=Inherit: Inherit via back propagation  NCopyOutMin=[]  NCopyOutMax=[]  IntegratorContinuousStateAttributes=''  IntegratorStateMustResolveToSignalObject=off  IntegratorRTWStateStorageClass=Auto  FilterContinuousStateAttributes=''  FilterStateMustResolveToSignalObject=off  FilterRTWStateStorageClass=Auto  ParallelPVariant=InternalParameters  IdealPVariant=Disabled  IVariant=InternalParameters  DVariant=InternalParameters  IntegratorVariant=Continuous  SatVariant=Disabled  AWVariant=Passthrough  PCopyVariant=Disabled  TRVariant=Disabled  FdbkBlocksVariant=Forward  IdealPFdbkVariant=Disabled  SatFdbkVariant=Disabled  DerivativeFilterVariant=ContFilter  NVariant=InternalParameters  NCopyVariant=Disabled  FilterICVariant=InternalICsFilter  IntegratorICVariant=InternalICs  ExternalResetVariant=Disabled  TRSumVariant=Passthrough  SumFdbkVariant=Disabled  SumVariant=Sum_PID  TsampFilterVariant=InternalTs  TsampNgainVariant=Passthrough  TsampIntegralVariant=Disabled_SignalSpec  ExternalSaturationOutDataTypeStr=Inherit: Same as second input  DerivativeSourceVariant=ErrorSignal  PreIntVariant=InternalPreInt
  Sin : Trigonometry
  Sum{,1..6,8,12..13,18,21..23} (14 alike) : Sum  Inputs=|+-
  Sum{7,10..11,14..15,17,19} (7 alike) : Sum  Inputs=|++
  "Thrust " : slpidlib/PID Controller  Controller=PID  Form=Parallel  TimeDomain=Continuous-time  UseExternalTs=off  SampleTime=-1  IntegratorMethod=Forward Euler  FilterMethod=Forward Euler  ControllerParametersSource=internal  P=1  I=1  UseKiTs=off  D=0  UseExternalDerivativeSource=off  N=100  UseFilter=on  TunerSelectOption=Transfer Function Based (PID Tuner App)  InitialConditionSource=internal  InitialConditionForIntegrator=0  InitialConditionForFilter=0  DifferentiatorICPrevScaledInput=0  ExternalReset=none  TrackingMode=off  Kt=1  LimitOutput=off  SatLimitsSource=internal  UpperSaturationLimit=inf  LowerSaturationLimit=-inf  LinearizeAsGain=on  AntiWindupMode=none  Kb=1  LimitIntegrator=off  UpperIntegratorSaturationLimit=inf  LowerIntegratorSaturationLimit=-inf  POutMin=[]  POutMax=[]  IOutMin=[]  IOutMax=[]  DOutMin=[]  DOutMax=[]  NOutMin=[]  NOutMax=[]  SumOutMin=[]  SumOutMax=[]  SaturationOutMin=[]  SaturationOutMax=[]  PParamMin=[]  PParamMax=[]  IParamMin=[]  IParamMax=[]  DParamMin=[]  DParamMax=[]  NParamMin=[]  NParamMax=[]  KbParamMin=[]  KbParamMax=[]  KtParamMin=[]  KtParamMax=[]  KbOutMin=[]  KbOutMax=[]  KtOutMin=[]  KtOutMax=[]  IntegratorOutMin=[]  IntegratorOutMax=[]  FilterOutMin=[]  FilterOutMax=[]  SumI1OutMin=[]  SumI1OutMax=[]  SumI2OutMin=[]  SumI2OutMax=[]  SumI3OutMin=[]  SumI3OutMax=[]  SumI4OutMin=[]  SumI4OutMax=[]  SumDOutMin=[]  SumDOutMax=[]  DifferentiatorOutMin=[]  DifferentiatorOutMax=[]  FilterDiffOutCoefMin=[]  FilterDiffOutCoefMax=[]  ReciprocalOutMin=[]  ReciprocalOutMax=[]  SumDenOutMin=[]  SumDenOutMax=[]  SumNumOutMin=[]  SumNumOutMax=[]  DivideOutMin=[]  DivideOutMax=[]  UdiffTsProdOutMin=[]  UdiffTsProdOutMax=[]  NTsProdOutMin=[]  NTsProdOutMax=[]  UintegralTsProdOutMin=[]  UintegralTsProdOutMax=[]  UngainTsProdOutMin=[]  UngainTsProdOutMax=[]  ClampingZeroOutDataTypeStr=Inherit: Inherit via back propagation  ClampingZeroOutMin=[]  ClampingZeroOutMax=[]  FilterDenConstantOutDataTypeStr=Inherit: Inherit via back propagation  FilterDenConstantOutMin=[]  FilterDenConstantOutMax=[]  PCopyOutDataTypeStr=Inherit: Inherit via back propagation  PCopyOutMin=[]  PCopyOutMax=[]  NCopyOutDataTypeStr=Inherit: Inherit via back propagation  NCopyOutMin=[]  NCopyOutMax=[]  IntegratorContinuousStateAttributes=''  IntegratorStateMustResolveToSignalObject=off  IntegratorRTWStateStorageClass=Auto  FilterContinuousStateAttributes=''  FilterStateMustResolveToSignalObject=off  FilterRTWStateStorageClass=Auto  ParallelPVariant=InternalParameters  IdealPVariant=Disabled  IVariant=InternalParameters  DVariant=InternalParameters  IntegratorVariant=Continuous  SatVariant=Disabled  AWVariant=Passthrough  PCopyVariant=Disabled  TRVariant=Disabled  FdbkBlocksVariant=Forward  IdealPFdbkVariant=Disabled  SatFdbkVariant=Disabled  DerivativeFilterVariant=ContFilter  NVariant=InternalParameters  NCopyVariant=Disabled  FilterICVariant=InternalICsFilter  IntegratorICVariant=InternalICs  ExternalResetVariant=Disabled  TRSumVariant=Passthrough  SumFdbkVariant=Disabled  SumVariant=Sum_PID  TsampFilterVariant=InternalTs  TsampNgainVariant=Passthrough  TsampIntegralVariant=Disabled_SignalSpec  ExternalSaturationOutDataTypeStr=Inherit: Same as second input  DerivativeSourceVariant=ErrorSignal  PreIntVariant=InternalPreInt
  "Yaw " : slpidlib/PID Controller  Controller=PID  Form=Parallel  TimeDomain=Continuous-time  UseExternalTs=off  SampleTime=-1  IntegratorMethod=Forward Euler  FilterMethod=Forward Euler  ControllerParametersSource=internal  P=1  I=1  UseKiTs=off  D=0  UseExternalDerivativeSource=off  N=100  UseFilter=on  TunerSelectOption=Transfer Function Based (PID Tuner App)  InitialConditionSource=internal  InitialConditionForIntegrator=0  InitialConditionForFilter=0  DifferentiatorICPrevScaledInput=0  ExternalReset=none  TrackingMode=off  Kt=1  LimitOutput=off  SatLimitsSource=internal  UpperSaturationLimit=inf  LowerSaturationLimit=-inf  LinearizeAsGain=on  AntiWindupMode=none  Kb=1  LimitIntegrator=off  UpperIntegratorSaturationLimit=inf  LowerIntegratorSaturationLimit=-inf  POutMin=[]  POutMax=[]  IOutMin=[]  IOutMax=[]  DOutMin=[]  DOutMax=[]  NOutMin=[]  NOutMax=[]  SumOutMin=[]  SumOutMax=[]  SaturationOutMin=[]  SaturationOutMax=[]  PParamMin=[]  PParamMax=[]  IParamMin=[]  IParamMax=[]  DParamMin=[]  DParamMax=[]  NParamMin=[]  NParamMax=[]  KbParamMin=[]  KbParamMax=[]  KtParamMin=[]  KtParamMax=[]  KbOutMin=[]  KbOutMax=[]  KtOutMin=[]  KtOutMax=[]  IntegratorOutMin=[]  IntegratorOutMax=[]  FilterOutMin=[]  FilterOutMax=[]  SumI1OutMin=[]  SumI1OutMax=[]  SumI2OutMin=[]  SumI2OutMax=[]  SumI3OutMin=[]  SumI3OutMax=[]  SumI4OutMin=[]  SumI4OutMax=[]  SumDOutMin=[]  SumDOutMax=[]  DifferentiatorOutMin=[]  DifferentiatorOutMax=[]  FilterDiffOutCoefMin=[]  FilterDiffOutCoefMax=[]  ReciprocalOutMin=[]  ReciprocalOutMax=[]  SumDenOutMin=[]  SumDenOutMax=[]  SumNumOutMin=[]  SumNumOutMax=[]  DivideOutMin=[]  DivideOutMax=[]  UdiffTsProdOutMin=[]  UdiffTsProdOutMax=[]  NTsProdOutMin=[]  NTsProdOutMax=[]  UintegralTsProdOutMin=[]  UintegralTsProdOutMax=[]  UngainTsProdOutMin=[]  UngainTsProdOutMax=[]  ClampingZeroOutDataTypeStr=Inherit: Inherit via back propagation  ClampingZeroOutMin=[]  ClampingZeroOutMax=[]  FilterDenConstantOutDataTypeStr=Inherit: Inherit via back propagation  FilterDenConstantOutMin=[]  FilterDenConstantOutMax=[]  PCopyOutDataTypeStr=Inherit: Inherit via back propagation  PCopyOutMin=[]  PCopyOutMax=[]  NCopyOutDataTypeStr=Inherit: Inherit via back propagation  NCopyOutMin=[]  NCopyOutMax=[]  IntegratorContinuousStateAttributes=''  IntegratorStateMustResolveToSignalObject=off  IntegratorRTWStateStorageClass=Auto  FilterContinuousStateAttributes=''  FilterStateMustResolveToSignalObject=off  FilterRTWStateStorageClass=Auto  ParallelPVariant=InternalParameters  IdealPVariant=Disabled  IVariant=InternalParameters  DVariant=InternalParameters  IntegratorVariant=Continuous  SatVariant=Disabled  AWVariant=Passthrough  PCopyVariant=Disabled  TRVariant=Disabled  FdbkBlocksVariant=Forward  IdealPFdbkVariant=Disabled  SatFdbkVariant=Disabled  DerivativeFilterVariant=ContFilter  NVariant=InternalParameters  NCopyVariant=Disabled  FilterICVariant=InternalICsFilter  IntegratorICVariant=InternalICs  ExternalResetVariant=Disabled  TRSumVariant=Passthrough  SumFdbkVariant=Disabled  SumVariant=Sum_PID  TsampFilterVariant=InternalTs  TsampNgainVariant=Passthrough  TsampIntegralVariant=Disabled_SignalSpec  ExternalSaturationOutDataTypeStr=Inherit: Same as second input  DerivativeSourceVariant=ErrorSignal  PreIntVariant=InternalPreInt
  Yaw_ref : Constant  Value=0
  x_net * cos(psi) : Product
  x_net * sin(psi) : Product
  x_ref : Constant  Value=0
  y_net * cos(psi) : Product
  y_net * sin(psi) : Product
  y_ref : Constant  Value=0
  z_ref : Constant  Value=0
  Motor Cmd : Outport
  wires:
  Cos/1 -> y_net * sin(psi)/2, y_net * cos(psi)/2
  Sum10/1 -> Sum11/1
  Sin/1 -> x_net * sin(psi)/1, x_net * cos(psi)/2
  y_net * sin(psi)/1 -> Sum6/2
  y_net * cos(psi)/1 -> Sum7/2
  x_net * sin(psi)/1 -> Sum6/1
  x_net * cos(psi)/1 -> Sum7/1
  "Pitch "/1 -> Sum22/2, Sum14/2, Sum18/2, Sum11/2
  Sum11/1 -> Sum12/1
  Demux/2 -> Sum1/2
  Sum17/1 -> Sum18/1
  Sum13/1 -> Sum14/1
  Sum21/1 -> Sum22/1
  AC Cmd/1 -> Bus Selector/1
  Sum18/1 -> Sum19/1
  Sum14/1 -> Sum15/1
  Sum22/1 -> Sum23/1
  z_ref/1 -> Sum8/1
  x_ref/1 -> Sum/1
  y_ref/1 -> Sum1/1
  Sum/1 -> x_net * cos(psi)/1, x_net * sin(psi)/2
  Sum1/1 -> y_net * cos(psi)/1, y_net * sin(psi)/1
  Sum8/1 -> Sum5/2
  PID Controller4/1 -> Sum2/2  "roll angle"
  PID Controller5/1 -> Sum3/2  "pitch angle"
  Yaw_ref/1 -> Sum4/1
  "Yaw "/1 -> Sum23/2, Sum19/2, Sum12/2, Sum15/2
  Sum4/1 -> "Yaw "/1  "Yaw"
  Sum3/1 -> "Pitch "/1  "Pitch"
  Roll/1 -> Sum10/2, Sum17/2, Sum21/2, Sum13/2
  "Thrust "/1 -> Sum13/1, Sum21/1, Sum10/1, Sum17/1
  Sum6/1 -> PID Controller4/1
  Sum7/1 -> PID Controller5/1
  Sum19/1 -> M3/1
  Sum15/1 -> M2/1
  Sum23/1 -> M4/1
  Sum12/1 -> M1/1
  Bus Selector/1 -> Sum4/2  "<YAW>"
  Sum2/1 -> Roll/1  "Roll"
  Sum5/1 -> "Thrust "/1  "Thrust"
  M1/1 -> Bus Creator/1  "M1"
  M3/1 -> Bus Creator/2  "M3"
  M2/1 -> Bus Creator/3  "M2"
  M4/1 -> Bus Creator/4  "M4"
  Bus Creator/1 -> Motor Cmd/1
  Sense/1 -> Bus Selector1/1
  Bus Selector1/1 -> Demux/1  "<pos_e>"
  Demux/1 -> Sum/2
  Demux/3 -> Sum8/2
  Bus Selector1/2 -> Bus Selector2/1  "<Yaw stuff>"
  Bus Selector2/1 -> Bus Creator/5  "<theta>"
  Bus Selector2/2 -> Cos/1, Sin/1  "<Yaw or psi>"
  Bus Selector2/3 -> Bus Creator/6  "<phi>"
  Bus Selector/2 -> Sum3/1  "<Pitch>"
  Bus Selector/3 -> Sum2/1  "<Roll>"
  Bus Selector/4 -> Sum5/1  "<Thrust>"

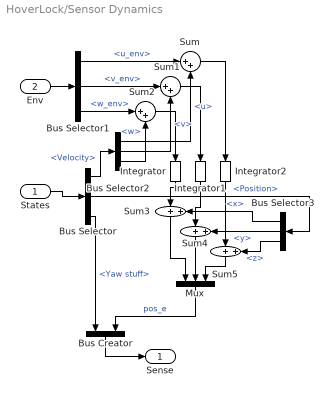
== system HoverLock/Sensor Dynamics ==
  States : Inport
  Env : Inport  Port=2
  Bus Creator : BusCreator  Inputs=2
  Bus Selector : BusSelector  OutputSignals=Velocity,Position,Yaw stuff
  Bus Selector1 : BusSelector  OutputSignals=u_env,v_env,w_env
  Bus Selector2 : BusSelector  OutputSignals=u,v,w
  Bus Selector3 : BusSelector  OutputSignals=x,y,z
  Integrator : Integrator
  Integrator1 : Integrator
  Integrator2 : Integrator
  Mux : Mux  Inputs=3
  Sum{,1..5} (6 alike) : Sum  Inputs=|++
  Sense : Outport
  wires:
  Bus Creator/1 -> Sense/1
  States/1 -> Bus Selector/1
  Bus Selector/1 -> Bus Selector2/1  "<Velocity>"
  Env/1 -> Bus Selector1/1
  Bus Selector1/1 -> Sum/1  "<u_env>"
  Bus Selector2/1 -> Sum/2  "<u>"
  Bus Selector1/2 -> Sum1/1  "<v_env>"
  Bus Selector2/2 -> Sum1/2  "<v>"
  Bus Selector1/3 -> Sum2/1  "<w_env>"
  Bus Selector2/3 -> Sum2/2  "<w>"
  Sum2/1 -> Integrator/1
  Sum1/1 -> Integrator1/1
  Sum/1 -> Integrator2/1
  Bus Selector/2 -> Bus Selector3/1  "<Position>"
  Integrator/1 -> Sum3/1
  Bus Selector3/1 -> Sum3/2  "<x>"
  Integrator1/1 -> Sum4/1
  Bus Selector3/2 -> Sum4/2  "<y>"
  Integrator2/1 -> Sum5/1
  Bus Selector3/3 -> Sum5/2  "<z>"
  Sum3/1 -> Mux/1
  Sum4/1 -> Mux/2
  Sum5/1 -> Mux/3
  Mux/1 -> Bus Creator/2  "pos_e"
  Bus Selector/3 -> Bus Creator/1  "<Yaw stuff>"

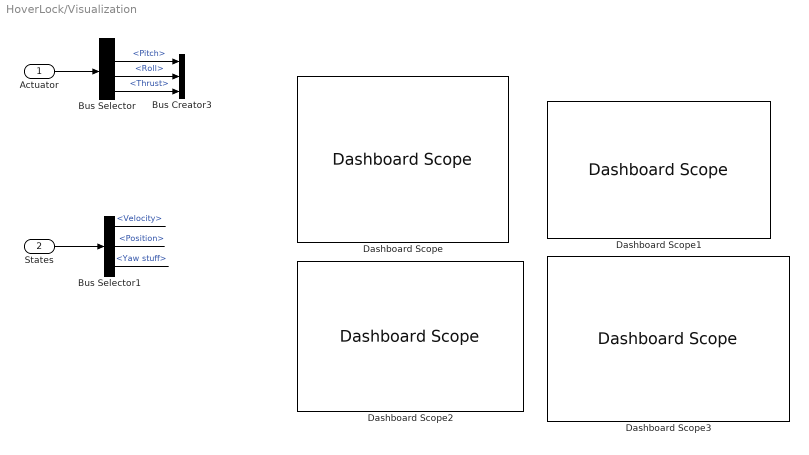
== system HoverLock/Visualization ==
  Actuator : Inport
  States : Inport  Port=2
  Bus Creator3 : BusCreator  Inputs=3
  Bus Selector : BusSelector  OutputSignals=YAW,Pitch,Roll,Thrust
  Bus Selector1 : BusSelector  OutputSignals=Velocity,Position,Yaw stuff
  Dashboard Scope{,1..3} (4 alike) : DashboardScope
  wires:
  Actuator/1 -> Bus Selector/1
  Bus Selector/3 -> Bus Creator3/2  "<Roll>"
  Bus Selector/4 -> Bus Creator3/3  "<Thrust>"
  States/1 -> Bus Selector1/1
  Bus Selector1/2 -> ?  "<Position>"
  Bus Selector1/3 -> ?  "<Yaw stuff>"
  Bus Selector1/1 -> ?  "<Velocity>"
  Bus Selector/2 -> Bus Creator3/1  "<Pitch>"

== matlab function HoverLock/Airframe/MATLAB Function1 ==
  data: p input; phi_dot output; q input; r input; phi input; theta input; theta_dot output; psi_dot output
function [phi_dot, theta_dot, psi_dot] = rates2euler(p, q, r, phi, theta)
phi_dot = p + sin(phi)*tan(theta)*q + cos(phi)*tan(theta)*r;
theta_dot = cos(phi)*q - sin(phi)*r;
psi_dot = (sin(phi)/cos(theta))*q + (cos(phi)/cos(theta))*r;
end

== matlab function HoverLock/Airframe/MATLAB Function ==
  data: phi input; R output; theta input; psi input
function R = rotMatrix(phi, theta, psi)

c_phi = cos(phi); s_phi = sin(phi);
c_theta = cos(theta); s_theta = sin(theta);
c_psi = cos(psi); s_psi = sin(psi);
R = [c_psi*c_theta, c_psi*s_theta*s_phi - s_psi*c_phi, c_psi*s_theta*c_phi + s_psi*s_phi;
     s_psi*c_theta, s_psi*s_theta*s_phi + c_psi*c_phi, s_psi*s_theta*c_phi - c_psi*s_phi;
     -s_theta, c_theta*s_phi, c_theta*c_phi];
end
